simulink model "P2_model"  (R2025b)
settings: Solver=ode4  StartTime=0.0  StopTime=3  FixedStep=20e-6  RelTol=1e-3
model workspace (MATLAB code in the model file):
  | Jw   = 1.2;   r = 0.30;
  | Jn   = 1.2;   lam = 20;   Ts = 1e-3;   Tmax = 600;
  | mode = 1;     zeta = 0.7; wa = 100;
  | quant_on = 0; act_on = 0; tau_act = 5e-3;
  | ka_conv = Jn^2*lam^2/(4*zeta^2);
  | ka      = wa*Ts;
undefined symbols (not defined in the file or in its folder): DiscIntNeverNeededParam
libraries: simulink x4
settings Model: Creator=Owner  LastModifiedBy=Owner

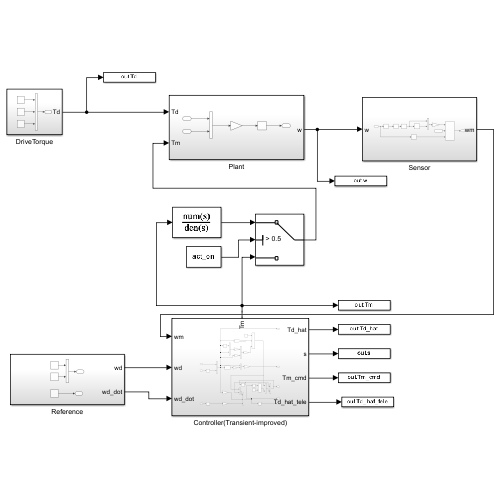
[thumbnail: Simulink's stored preview of the top-level diagram]
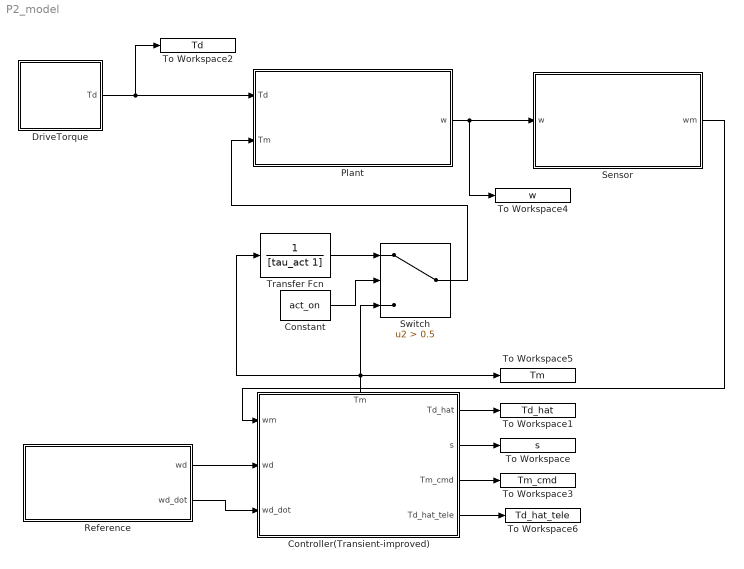
== system P2_model ==
  Constant : Constant  Value=act_on
  Controller(Transient-improved) : Subsystem
      settings: PortSchema="{\"entries\":[{\"content\":{\"sides\":[{\"content\":{\"connectorIds\":[\"In1\",\"In2\",\"In3\"]},\"type\":\"ConnectorPlacement.EquallySpacedRectSide\",\"uuid\":\"db018cbb-f712-44f0-9512-4d94f82516be\"},{\"content\":{\"connectorIds\":[\"Out1\",\"Out2\",\"Out3\",\"Out4\"],\"side\":\"RIGHT\"},\"type\":\"ConnectorPlacement.EquallySpacedRectSide\",\"uuid\":\"79f58bb9-febf-4414-88b5-61586d37b576\"},{\"content\":{\"connectorIds\":[\"Out5\"],\"side\":\"TOP\"},\"type\":\"ConnectorPlacement.EquallySpacedRectSide\",\"uuid\":\"ac911475-5310-46a2-bcdf-979d5982e8b1\"}]},\"type\":\"ConnectorPlacement.EquallySpacedConnector\",\"uuid\":\"5be97a90-a621-4e93-a7ea-194a2e1030e6\"}],\"packageUris\":[\"http://schema.mathworks.com/mf0/Connector/R2020b\"],\"version\":\"1.0\"}"
  DriveTorque : Subsystem
  Plant : Subsystem
  Reference : Subsystem
  Sensor : Subsystem
  Switch : Switch  Criteria=u2 > Threshold  Threshold=0.5  SaturateOnIntegerOverflow=off  InputSameDT=off
  To Workspace : ToWorkspace  VariableName=s  SaveFormat=Timeseries  SampleTime=-1
  To Workspace1 : ToWorkspace  VariableName=Td_hat  SaveFormat=Timeseries  SampleTime=-1
  To Workspace2 : ToWorkspace  VariableName=Td  SaveFormat=Timeseries  SampleTime=-1
  To Workspace3 : ToWorkspace  VariableName=Tm_cmd  SaveFormat=Timeseries  SampleTime=-1
  To Workspace4 : ToWorkspace  VariableName=w  SaveFormat=Timeseries  SampleTime=-1
  To Workspace5 : ToWorkspace  VariableName=Tm  SaveFormat=Timeseries  SampleTime=-1
  To Workspace6 : ToWorkspace  VariableName=Td_hat_tele  SaveFormat=Timeseries  SampleTime=-1
  Transfer Fcn : TransferFcn  Denominator=[tau_act 1]
  wires:
  Plant/1(w) -> To Workspace4/1, Sensor/1(w)
  Reference/1(wd) -> Controller(Transient-improved)/2(wd)
  Reference/2(wd_dot) -> Controller(Transient-improved)/3(wd_dot)
  Controller(Transient-improved)/5(Tm) -> Switch/3, Transfer Fcn/1, To Workspace5/1
  Controller(Transient-improved)/2(s) -> To Workspace/1
  Controller(Transient-improved)/1(Td_hat) -> To Workspace1/1
  Controller(Transient-improved)/3(Tm_cmd) -> To Workspace3/1
  Controller(Transient-improved)/4(Td_hat_tele) -> To Workspace6/1
  DriveTorque/1(Td) -> To Workspace2/1, Plant/1(Td)
  Transfer Fcn/1 -> Switch/1
  Constant/1 -> Switch/2
  Switch/1 -> Plant/2(Tm)
  Sensor/1(wm) -> Controller(Transient-improved)/1(wm)

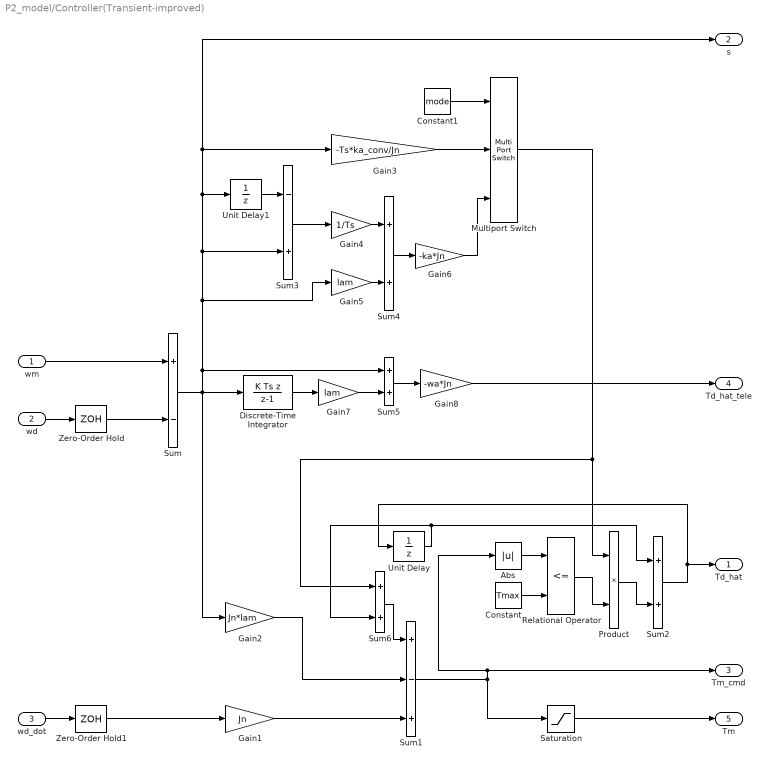
== system P2_model/Controller(Transient-improved) ==
  wm : Inport
  wd : Inport  Port=2
  wd_dot : Inport  Port=3
  Abs : Abs  SaturateOnIntegerOverflow=off
  Constant : Constant  Value=Tmax
  Constant1 : Constant  Value=mode
  Discrete-Time Integrator : DiscreteIntegrator  IntegratorMethod=Integration: Backward Euler  SampleTime=Ts  ICPrevOutput=DiscIntNeverNeededParam  ICPrevScaledInput=DiscIntNeverNeededParam
  Gain1 : Gain  Gain=Jn
  Gain2 : Gain  Gain=Jn*lam
  Gain3 : Gain  Gain=-Ts*ka_conv/Jn
  Gain4 : Gain  Gain=1/Ts
  Gain5 : Gain  Gain=lam
  Gain6 : Gain  Gain=-ka*Jn
  Gain7 : Gain  Gain=lam
  Gain8 : Gain  Gain=-wa*Jn
  Multiport Switch : MultiPortSwitch  Inputs=2  SaturateOnIntegerOverflow=off  InputSameDT=off
  Product : Product
  Relational Operator : RelationalOperator  Operator=<=  OutDataTypeStr=boolean  RndMeth=Simplest  InputSameDT=off
  Saturation : Saturate  UpperLimit=Tmax  LowerLimit=-Tmax
  Sum : Sum  Inputs=+-
  Sum1 : Sum  Inputs=+-+
  Sum{2,4..6} (4 alike) : Sum
  Sum3 : Sum  Inputs=-+
  Unit Delay : UnitDelay  SampleTime=Ts  HasFrameUpgradeWarning=on
  Unit Delay1 : UnitDelay  SampleTime=Ts  HasFrameUpgradeWarning=on
  Zero-Order Hold : ZeroOrderHold  SampleTime=Ts
  Zero-Order Hold1 : ZeroOrderHold  SampleTime=Ts
  Td_hat : Outport
  s : Outport  Port=2
  Tm_cmd : Outport  Port=3
  Td_hat_tele : Outport  Port=4
  Tm : Outport  Port=5
  wires:
  wd/1 -> Zero-Order Hold/1
  wd_dot/1 -> Zero-Order Hold1/1
  Zero-Order Hold/1 -> Sum/2
  wm/1 -> Sum/1
  Sum/1 -> Gain2/1, Discrete-Time Integrator/1, s/1, Gain3/1, Unit Delay1/1, Sum3/2, Gain5/1, Sum5/1
  Sum1/1 -> Abs/1, Tm_cmd/1, Saturation/1
  Zero-Order Hold1/1 -> Gain1/1
  Gain1/1 -> Sum1/3
  Saturation/1 -> Tm/1
  Gain2/1 -> Sum1/2
  Constant/1 -> Relational Operator/2
  Abs/1 -> Relational Operator/1
  Relational Operator/1 -> Product/2
  Product/1 -> Sum2/2
  Sum2/1 -> Td_hat/1, Unit Delay/1
  Unit Delay/1 -> Sum6/2, Sum2/1
  Unit Delay1/1 -> Sum3/1
  Sum3/1 -> Gain4/1
  Gain4/1 -> Sum4/1
  Gain5/1 -> Sum4/2
  Sum4/1 -> Gain6/1
  Gain3/1 -> Multiport Switch/2
  Gain6/1 -> Multiport Switch/3
  Constant1/1 -> Multiport Switch/1
  Multiport Switch/1 -> Sum6/1, Product/1
  Discrete-Time Integrator/1 -> Gain7/1
  Gain7/1 -> Sum5/2
  Sum5/1 -> Gain8/1
  Gain8/1 -> Td_hat_tele/1
  Sum6/1 -> Sum1/1

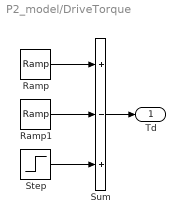
== system P2_model/DriveTorque ==
  Ramp : simulink/Sources/Ramp  slope=1500  start=0.5  InitialOutput=0
  Ramp1 : simulink/Sources/Ramp  slope=1500  start=0.7  InitialOutput=0
  Step : Step  Time=1.5  After=-180  SampleTime=0
  Sum : Sum  Inputs=+-+
  Td : Outport
  wires:
  Ramp/1 -> Sum/1
  Ramp1/1 -> Sum/2
  Step/1 -> Sum/3
  Sum/1 -> Td/1

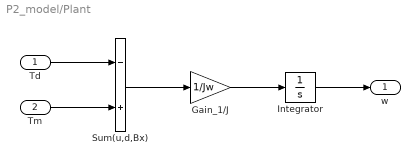
== system P2_model/Plant ==
  Td : Inport
  Tm : Inport  Port=2
  Gain_1/J : Gain  Gain=1/Jw
  Integrator : Integrator
  Sum(u,d,Bx) : Sum  Inputs=-+
  w : Outport
  wires:
  Tm/1 -> Sum(u,d,Bx)/2
  Sum(u,d,Bx)/1 -> Gain_1/J/1
  Gain_1/J/1 -> Integrator/1
  Integrator/1 -> w/1
  Td/1 -> Sum(u,d,Bx)/1

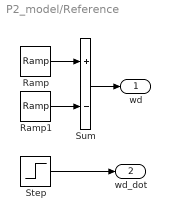
== system P2_model/Reference ==
  Ramp : simulink/Sources/Ramp  slope=20  start=0  InitialOutput=0
  Ramp1 : simulink/Sources/Ramp  slope=20  start=2  InitialOutput=0
  Step : Step  Time=2  Before=20  After=0  SampleTime=0
  Sum : Sum  Inputs=+-
  wd : Outport
  wd_dot : Outport  Port=2
  wires:
  Ramp/1 -> Sum/1
  Ramp1/1 -> Sum/2
  Sum/1 -> wd/1
  Step/1 -> wd_dot/1

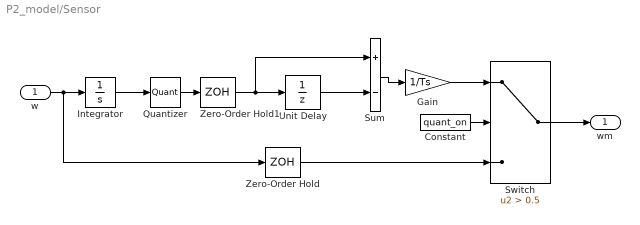
== system P2_model/Sensor ==
  w : Inport
  Constant : Constant  Value=quant_on
  Gain : Gain  Gain=1/Ts
  Integrator : Integrator
  Quantizer : Quantizer  QuantizationInterval=2*pi/4096
  Sum : Sum  Inputs=+-
  Switch : Switch  Criteria=u2 > Threshold  Threshold=0.5  SaturateOnIntegerOverflow=off  InputSameDT=off
  Unit Delay : UnitDelay  SampleTime=Ts  HasFrameUpgradeWarning=on
  Zero-Order Hold : ZeroOrderHold  SampleTime=Ts
  Zero-Order Hold1 : ZeroOrderHold  SampleTime=Ts
  wm : Outport
  wires:
  Zero-Order Hold1/1 -> Sum/1, Unit Delay/1
  w/1 -> Zero-Order Hold/1, Integrator/1
  Integrator/1 -> Quantizer/1
  Quantizer/1 -> Zero-Order Hold1/1
  Unit Delay/1 -> Sum/2
  Sum/1 -> Gain/1
  Gain/1 -> Switch/1
  Constant/1 -> Switch/2
  Zero-Order Hold/1 -> Switch/3
  Switch/1 -> wm/1
